simulink model "HW2"  (R2022b)
settings: Solver=VariableStepAuto  StartTime=0.0  StopTime=50  RelTol=1e-3
settings Model: Creator=ali14  LastModifiedBy=ali14

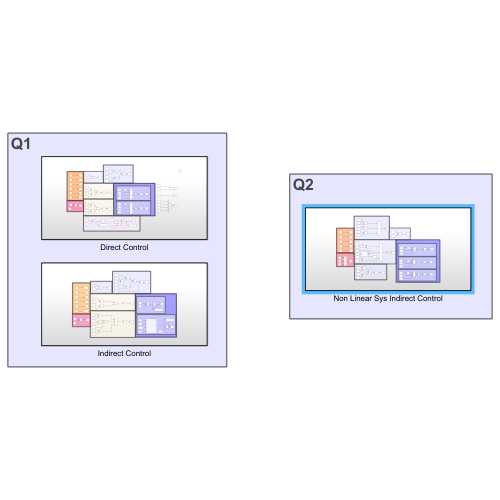
[thumbnail: Simulink's stored preview of the top-level diagram]
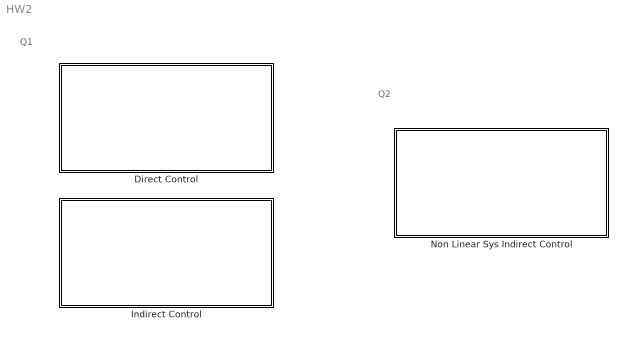
== system HW2 ==
  note: Q2
  note: Q1
  Direct Control : Subsystem
  Indirect Control : Subsystem
  Non Linear Sys Indirect Control : Subsystem

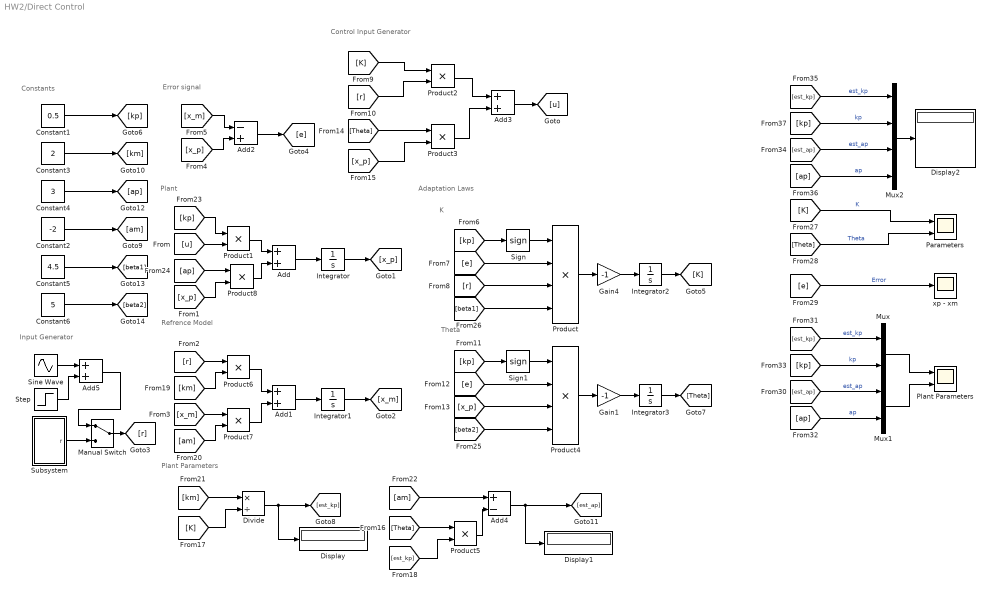
== system HW2/Direct Control ==
  note: Plant Parameters
  note: Input Generator
  note: Control Input Generator
  note: Constants
  note: Adaptation Laws
  note: Theta
  note: K
  note: Refrence Model
  note: Error signal
  note: Plant
  Add{,1,3,5} (4 alike) : Sum
  Add2 : Sum  Inputs=-+
  Add4 : Sum  Inputs=+-
  Constant1 : Constant  Value=0.5
  Constant2 : Constant  Value=-2
  Constant3 : Constant  Value=2
  Constant4 : Constant  Value=3
  Constant5 : Constant  Value=4.5
  Constant6 : Constant  Value=5
  Display : Display
  Display1 : Display
  Display2 : Display
  Divide : Product  Inputs=*/
  Gain1 : Gain  Gain=-1
  Gain4 : Gain  Gain=-1
  Integrator{,1..3} (4 alike) : Integrator
  Manual Switch : ManualSwitch
  Mux : Mux  Inputs=2
  Mux1 : Mux  Inputs=2
  Mux2 : Mux
  Parameters : Scope  NumInputPorts=2
  Plant Parameters : Scope  NumInputPorts=2
  Product : Product  Inputs=4
  Product{1..3,5..8} (7 alike) : Product
  Product4 : Product  Inputs=4
  Sign : Signum
  Sign1 : Signum
  Sine Wave : Sin  Amplitude=3  Frequency=2  SampleTime=0
  Step : Step  SampleTime=0
  Subsystem : Subsystem
  xp - xm : Scope
  wires:
  Constant3/1 -> [km]
  [r] -> Product2/2
  Integrator2/1 -> [K]
  Constant1/1 -> [kp]
  Product1/1 -> Add/1
  Constant2/1 -> [am]
  Gain4/1 -> Integrator2/1
  [kp] -> Product1/1
  Add2/1 -> [e]
  Add5/1 -> Manual Switch/1
  [u] -> Product1/2
  Sign1/1 -> Product4/1
  [x_p] -> Product4/3
  [K] -> Product2/1
  Product3/1 -> Add3/2
  [x_p] -> Add2/2
  Add/1 -> Integrator/1
  [r] -> Product/3
  [e] -> Product/2
  [e] -> Product4/2
  Constant4/1 -> [ap]
  [km] -> Product6/2
  [kp] -> Sign1/1
  Add3/1 -> [u]
  Sign/1 -> Product/1
  Gain1/1 -> Integrator3/1
  Add1/1 -> Integrator1/1
  Product8/1 -> Add/2
  Integrator/1 -> [x_p]
  Product2/1 -> Add3/1
  [x_m] -> Add2/1
  [x_p] -> Product8/2
  Integrator1/1 -> [x_m]
  Product/1 -> Gain4/1
  [r] -> Product6/1
  Integrator3/1 -> [Theta]
  [x_p] -> Product3/2
  [ap] -> Product8/1
  [kp] -> Sign/1
  [Theta] -> Product3/1
  Step/1 -> Add5/2
  [x_m] -> Product7/1
  Product4/1 -> Gain1/1
  Product6/1 -> Add1/1
  Sine Wave/1 -> Add5/1
  [am] -> Product7/2
  Product7/1 -> Add1/2
  Divide/1 -> [est_kp], Display/1
  [km] -> Divide/1
  [K] -> Divide/2
  [am] -> Add4/1
  [est_kp] -> Product5/2
  Product5/1 -> Add4/2
  [Theta] -> Product5/1
  Add4/1 -> [est_ap], Display1/1
  Constant5/1 -> [beta1]
  Constant6/1 -> [beta2]
  [beta1] -> Product/4
  [beta2] -> Product4/4
  [K] -> Parameters/1  "K"
  [Theta] -> Parameters/2  "Theta"
  [e] -> xp - xm/1  "Error"
  [kp] -> Mux/2  "kp"
  [est_kp] -> Mux/1  "est_kp"
  [ap] -> Mux1/2  "ap"
  [est_ap] -> Mux1/1  "est_ap"
  Mux/1 -> Plant Parameters/1
  Mux1/1 -> Plant Parameters/2
  [est_ap] -> Mux2/3  "est_ap"
  [ap] -> Mux2/4  "ap"
  [kp] -> Mux2/2  "kp"
  [est_kp] -> Mux2/1  "est_kp"
  Mux2/1 -> Display2/1
  Subsystem/1(r) -> Manual Switch/2
  Manual Switch/1 -> [r]

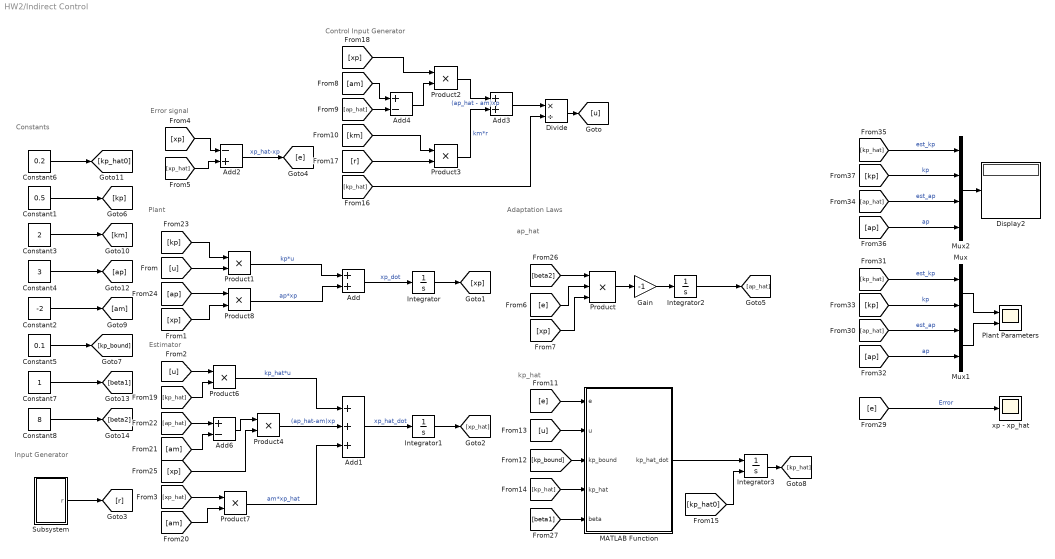
== system HW2/Indirect Control ==
  note: Input Generator
  note: Control Input Generator
  note: Constants
  note: Adaptation Laws
  note: kp_hat
  note: ap_hat
  note: Estimator
  note: Error signal
  note: Plant
  Add : Sum
  Add1 : Sum  Inputs=+++
  Add2 : Sum  Inputs=-+
  Add3 : Sum
  Add4 : Sum  Inputs=+-
  Add6 : Sum  Inputs=+-
  Constant1 : Constant  Value=0.5
  Constant2 : Constant  Value=-2
  Constant3 : Constant  Value=2
  Constant4 : Constant  Value=3
  Constant5 : Constant  Value=0.1
  Constant6 : Constant  Value=0.2
  Constant7 : Constant
  Constant8 : Constant  Value=8
  Display2 : Display
  Divide : Product  Inputs=*/
  Gain : Gain  Gain=-1
  Integrator : Integrator
  Integrator1 : Integrator
  Integrator2 : Integrator
  Integrator3 : Integrator  InitialConditionSource=external
  MATLAB Function : MATLAB Function  TreatAsAtomicUnit=on
  Mux : Mux  Inputs=2
  Mux1 : Mux  Inputs=2
  Mux2 : Mux
  Plant Parameters : Scope  NumInputPorts=2
  Product : Product  Inputs=3
  Product{1..4,6..8} (7 alike) : Product
  Subsystem : Subsystem
  xp - xp_hat : Scope
  wires:
  Constant3/1 -> [km]
  Constant1/1 -> [kp]
  Product1/1 -> Add/1  "kp*u"
  Constant2/1 -> [am]
  [kp] -> Product1/1
  Add2/1 -> [e]  "xp_hat-xp"
  [u] -> Product1/2
  Add/1 -> Integrator/1  "xp_dot"
  Constant4/1 -> [ap]
  [kp_hat] -> Product6/2
  Add1/1 -> Integrator1/1  "xp_hat_dot"
  Product8/1 -> Add/2  "ap*xp"
  Integrator/1 -> [xp]
  [xp] -> Add2/1
  [xp] -> Product8/2
  Integrator1/1 -> [xp_hat]
  [u] -> Product6/1
  [ap] -> Product8/1
  [xp_hat] -> Product7/1
  Product6/1 -> Add1/1  "kp_hat*u"
  [am] -> Product7/2
  Product/1 -> Gain/1
  Add3/1 -> Divide/1
  Divide/1 -> [u]
  [am] -> Add4/1
  [ap_hat] -> Add4/2
  Constant5/1 -> [kp_bound]
  Integrator2/1 -> [ap_hat]
  [e] -> MATLAB Function/1(e)
  [kp_bound] -> MATLAB Function/3(kp_bound)
  [u] -> MATLAB Function/2(u)
  MATLAB Function/1(kp_hat_dot) -> Integrator3/1
  Integrator3/1 -> [kp_hat]
  [kp_hat] -> MATLAB Function/4(kp_hat)
  Constant6/1 -> [kp_hat0]
  [kp_hat0] -> Integrator3/2
  [kp_hat] -> Divide/2
  [km] -> Product3/1
  Product3/1 -> Add3/2  "km*r"
  [r] -> Product3/2
  Add4/1 -> Product2/2
  Product2/1 -> Add3/1  "(ap_hat - am)xp"
  [xp] -> Product2/1
  Product7/1 -> Add1/3  "am*xp_hat"
  [am] -> Add6/2
  [ap_hat] -> Add6/1
  Add6/1 -> Product4/1
  Product4/1 -> Add1/2  "(ap_hat-am)xp"
  [xp] -> Product4/2
  [xp_hat] -> Add2/2
  [kp_hat] -> Mux2/1  "est_kp"
  [ap] -> Mux2/4  "ap"
  [kp] -> Mux2/2  "kp"
  Mux2/1 -> Display2/1
  [ap_hat] -> Mux2/3  "est_ap"
  [ap_hat] -> Mux1/1  "est_ap"
  Mux1/1 -> Plant Parameters/2
  [ap] -> Mux1/2  "ap"
  [kp] -> Mux/2  "kp"
  Mux/1 -> Plant Parameters/1
  [kp_hat] -> Mux/1  "est_kp"
  Constant8/1 -> [beta2]
  Constant7/1 -> [beta1]
  [beta2] -> Product/1
  [e] -> Product/2
  [xp] -> Product/3
  [beta1] -> MATLAB Function/5(beta)
  Subsystem/1(r) -> [r]
  [e] -> xp - xp_hat/1  "Error"
  Gain/1 -> Integrator2/1

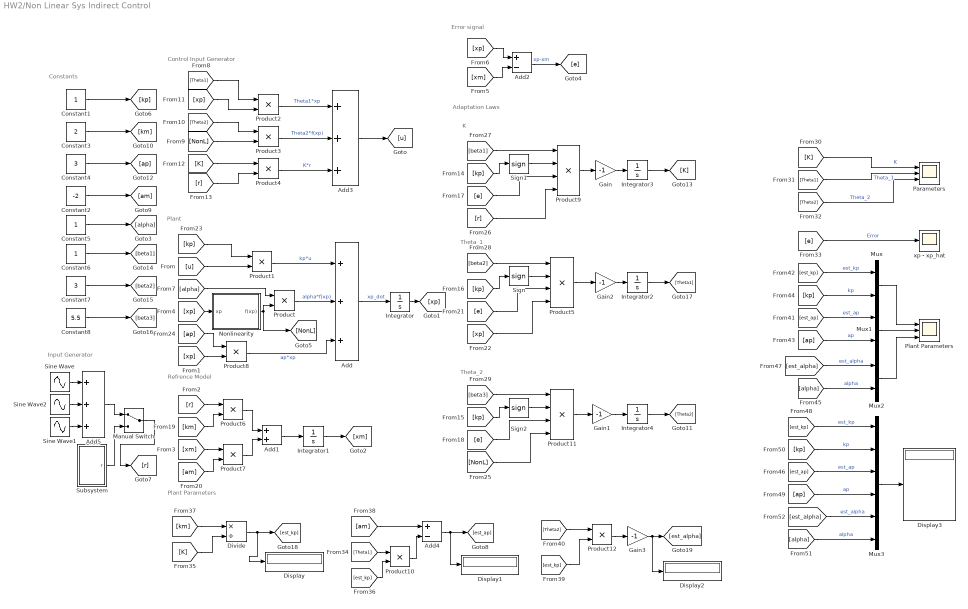
== system HW2/Non Linear Sys Indirect Control ==
  note: Theta_1
  note: Theta_2
  note: K
  note: Control Input Generator
  note: Adaptation Laws
  note: Refrence Model
  note: Plant
  note: Constants
  note: Error signal
  note: Input Generator
  note: Plant Parameters
  Add : Sum  Inputs=+++
  Add1 : Sum
  Add2 : Sum  Inputs=+-
  Add3 : Sum  Inputs=+++
  Add4 : Sum  Inputs=+-
  Add5 : Sum  Inputs=+++
  Constant1 : Constant
  Constant2 : Constant  Value=-2
  Constant3 : Constant  Value=2
  Constant4 : Constant  Value=3
  Constant5 : Constant
  Constant6 : Constant
  Constant7 : Constant  Value=3
  Constant8 : Constant  Value=5.5
  Display{,1..3} (4 alike) : Display
  Divide : Product  Inputs=*/
  Gain{,1..3} (4 alike) : Gain  Gain=-1
  Integrator{,1..4} (5 alike) : Integrator
  Manual Switch : ManualSwitch
  Mux : Mux  Inputs=2
  Mux1 : Mux  Inputs=2
  Mux2 : Mux  Inputs=2
  Mux3 : Mux  Inputs=6
  Nonlinearity : Subsystem
  Parameters : Scope  NumInputPorts=3
  Plant Parameters : Scope  NumInputPorts=3
  Product{,1..4,6..8,10,12} (10 alike) : Product
  Product11 : Product  Inputs=4
  Product5 : Product  Inputs=4
  Product9 : Product  Inputs=4
  Sign : Signum
  Sign1 : Signum
  Sign2 : Signum
  Sine Wave : Sin  Frequency=5  SampleTime=0
  Sine Wave1 : Sin  Frequency=10  SampleTime=0
  Sine Wave2 : Sin  Frequency=2  SampleTime=0
  Subsystem : Subsystem
  xp - xp_hat : Scope
  wires:
  Product7/1 -> Add1/2
  [xm] -> Product7/1
  [am] -> Product7/2
  Product6/1 -> Add1/1
  Add1/1 -> Integrator1/1
  [km] -> Product6/2
  Integrator1/1 -> [xm]
  [r] -> Product6/1
  [ap] -> Product8/1
  [xp] -> Product8/2
  Integrator/1 -> [xp]
  Add/1 -> Integrator/1  "xp_dot"
  [kp] -> Product1/1
  [u] -> Product1/2
  Product1/1 -> Add/1  "kp*u"
  Constant4/1 -> [ap]
  Constant1/1 -> [kp]
  Constant3/1 -> [km]
  Constant2/1 -> [am]
  Product8/1 -> Add/3  "ap*xp"
  [xp] -> Nonlinearity/1(xp)
  [xm] -> Add2/2
  [xp] -> Add2/1
  Add2/1 -> [e]  "xp-xm"
  Constant5/1 -> [alpha]
  Product/1 -> Add/2  "alpha*f(xp)"
  [alpha] -> Product/1
  Add3/1 -> [u]
  Product2/1 -> Add3/1  "Theta1*xp"
  [Theta1] -> Product2/1
  [xp] -> Product2/2
  Product3/1 -> Add3/2  "Theta2*f(xp)"
  Product4/1 -> Add3/3  "K*r"
  [K] -> Product4/1
  [NonL] -> Product3/2
  [Theta2] -> Product3/1
  Sine Wave2/1 -> Add5/2
  [r] -> Product4/2
  Nonlinearity/1(f(xp)) -> Product/2, [NonL]
  Integrator2/1 -> [Theta1]
  Integrator4/1 -> [Theta2]
  Product5/1 -> Gain2/1
  Product9/1 -> Gain/1
  Product11/1 -> Gain1/1
  [kp] -> Sign1/1
  [kp] -> Sign/1
  Integrator3/1 -> [K]
  Gain/1 -> Integrator3/1
  Gain1/1 -> Integrator4/1
  Gain2/1 -> Integrator2/1
  Sine Wave/1 -> Add5/1
  Sine Wave1/1 -> Add5/3
  Constant7/1 -> [beta2]
  Constant6/1 -> [beta1]
  Constant8/1 -> [beta3]
  Sign1/1 -> Product9/2
  [e] -> Product9/3
  [r] -> Product9/4
  [beta1] -> Product9/1
  [beta2] -> Product5/1
  Sign/1 -> Product5/2
  [e] -> Product5/3
  [xp] -> Product5/4
  [kp] -> Sign2/1
  Sign2/1 -> Product11/2
  [e] -> Product11/3
  [beta3] -> Product11/1
  [NonL] -> Product11/4
  [Theta1] -> Parameters/2  "Theta_1"
  [K] -> Parameters/1  "K"
  [Theta2] -> Parameters/3  "Theta_2"
  [e] -> xp - xp_hat/1  "Error"
  Add4/1 -> [est_ap], Display1/1
  [am] -> Add4/1
  [Theta1] -> Product10/1
  [km] -> Divide/1
  [est_kp] -> Product10/2
  Product10/1 -> Add4/2
  Divide/1 -> [est_kp], Display/1
  [K] -> Divide/2
  [est_kp] -> Product12/2
  [Theta2] -> Product12/1
  Product12/1 -> Gain3/1
  Gain3/1 -> Display2/1, [est_alpha]
  Mux1/1 -> Plant Parameters/2
  [est_kp] -> Mux/1  "est_kp"
  [ap] -> Mux1/2  "ap"
  [est_ap] -> Mux1/1  "est_ap"
  [kp] -> Mux/2  "kp"
  Mux/1 -> Plant Parameters/1
  [alpha] -> Mux2/2  "alpha"
  [est_alpha] -> Mux2/1  "est_alpha"
  Mux2/1 -> Plant Parameters/3
  [ap] -> Mux3/4  "ap"
  [est_kp] -> Mux3/1  "est_kp"
  [kp] -> Mux3/2  "kp"
  Mux3/1 -> Display3/1
  [est_ap] -> Mux3/3  "est_ap"
  [est_alpha] -> Mux3/5  "est_alpha"
  [alpha] -> Mux3/6  "alpha"
  Add5/1 -> Manual Switch/1
  Subsystem/1(r) -> Manual Switch/2
  Manual Switch/1 -> [r]

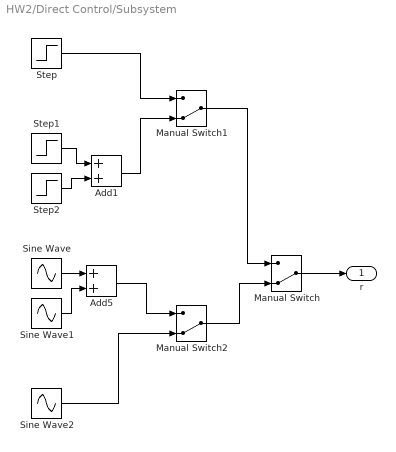
== system HW2/Direct Control/Subsystem ==
  Add1 : Sum
  Add5 : Sum
  Manual Switch : ManualSwitch  CurrentSetting=0
  Manual Switch1 : ManualSwitch  CurrentSetting=0
  Manual Switch2 : ManualSwitch  CurrentSetting=0
  Sine Wave : Sin  Amplitude=3  Frequency=2  SampleTime=0
  Sine Wave1 : Sin  Amplitude=2  Frequency=5  SampleTime=0
  Sine Wave2 : Sin  Amplitude=3  Frequency=2  SampleTime=0
  Step : Step  Time=0  SampleTime=0
  Step1 : Step  Time=0  SampleTime=0
  Step2 : Step  Time=0  SampleTime=0
  r : Outport
  wires:
  Sine Wave1/1 -> Add5/2
  Sine Wave/1 -> Add5/1
  Manual Switch/1 -> r/1
  Step/1 -> Manual Switch1/1
  Step1/1 -> Add1/1
  Step2/1 -> Add1/2
  Add1/1 -> Manual Switch1/2
  Manual Switch1/1 -> Manual Switch/1
  Sine Wave2/1 -> Manual Switch2/2
  Add5/1 -> Manual Switch2/1
  Manual Switch2/1 -> Manual Switch/2

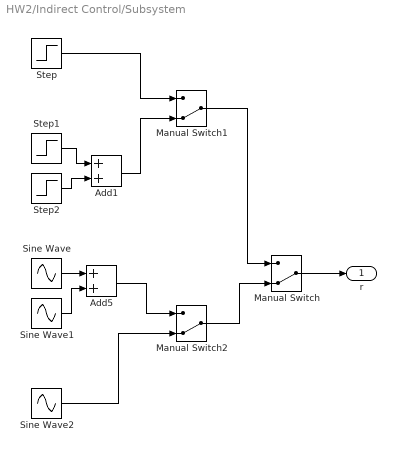
== system HW2/Indirect Control/Subsystem ==
  Add1 : Sum
  Add5 : Sum
  Manual Switch : ManualSwitch  CurrentSetting=0
  Manual Switch1 : ManualSwitch  CurrentSetting=0
  Manual Switch2 : ManualSwitch  CurrentSetting=0
  Sine Wave : Sin  Amplitude=3  Frequency=2  SampleTime=0
  Sine Wave1 : Sin  Amplitude=2  Frequency=5  SampleTime=0
  Sine Wave2 : Sin  Amplitude=3  Frequency=2  SampleTime=0
  Step : Step  Time=0  SampleTime=0
  Step1 : Step  Time=0  SampleTime=0
  Step2 : Step  Time=0  SampleTime=0
  r : Outport
  wires:
  Sine Wave1/1 -> Add5/2
  Sine Wave/1 -> Add5/1
  Manual Switch/1 -> r/1
  Step/1 -> Manual Switch1/1
  Step1/1 -> Add1/1
  Step2/1 -> Add1/2
  Add1/1 -> Manual Switch1/2
  Manual Switch1/1 -> Manual Switch/1
  Sine Wave2/1 -> Manual Switch2/2
  Add5/1 -> Manual Switch2/1
  Manual Switch2/1 -> Manual Switch/2

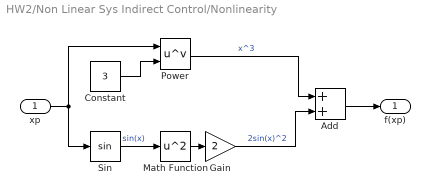
== system HW2/Non Linear Sys Indirect Control/Nonlinearity ==
  xp : Inport
  Add : Sum
  Constant : Constant  Value=3
  Gain : Gain  Gain=2
  Math Function : Math  Operator=square
  Power : Math  Operator=pow
  Sin : Trigonometry
  f(xp) : Outport
  wires:
  xp/1 -> Sin/1, Power/1
  Constant/1 -> Power/2
  Sin/1 -> Math Function/1  "sin(x)"
  Add/1 -> f(xp)/1
  Power/1 -> Add/1  "x^3"
  Math Function/1 -> Gain/1
  Gain/1 -> Add/2  "2sin(x)^2"

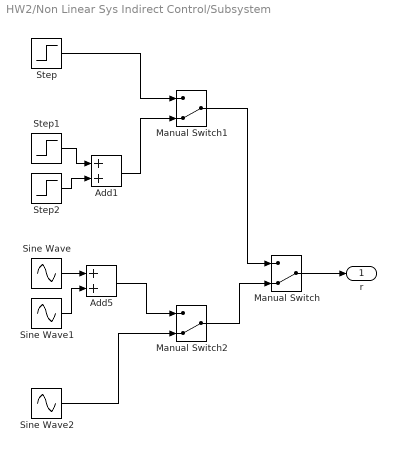
== system HW2/Non Linear Sys Indirect Control/Subsystem ==
  Add1 : Sum
  Add5 : Sum
  Manual Switch : ManualSwitch  CurrentSetting=0
  Manual Switch1 : ManualSwitch  CurrentSetting=0
  Manual Switch2 : ManualSwitch  CurrentSetting=0
  Sine Wave : Sin  Amplitude=3  Frequency=2  SampleTime=0
  Sine Wave1 : Sin  Amplitude=2  Frequency=5  SampleTime=0
  Sine Wave2 : Sin  Amplitude=3  Frequency=2  SampleTime=0
  Step : Step  Time=0  SampleTime=0
  Step1 : Step  Time=0  SampleTime=0
  Step2 : Step  Time=0  SampleTime=0
  r : Outport
  wires:
  Sine Wave1/1 -> Add5/2
  Sine Wave/1 -> Add5/1
  Manual Switch/1 -> r/1
  Step/1 -> Manual Switch1/1
  Step1/1 -> Add1/1
  Step2/1 -> Add1/2
  Add1/1 -> Manual Switch1/2
  Manual Switch1/1 -> Manual Switch/1
  Sine Wave2/1 -> Manual Switch2/2
  Add5/1 -> Manual Switch2/1
  Manual Switch2/1 -> Manual Switch/2

== matlab function HW2/Indirect Control/MATLAB Function ==
  data: e input; u input; kp_hat_dot output; kp_bound input; kp_hat input; beta input
function kp_hat_dot = fcn(e,u,kp_bound,kp_hat,beta)


if e*u <0
    kp_hat_dot = -beta*e*u;
else 
    if kp_hat > kp_bound
        kp_hat_dot = -beta*e*u;
    else 
        kp_hat_dot = 0;
    end
end
